simulink model "Trapezoidal_Commutation_BLDC_Motor_2024b"  (R2024b)
settings: Solver=VariableStepAuto  StartTime=0.0  StopTime=2  RelTol=1e-3
libraries: nesl_utility x11, ee_lib x10, fl_lib x6
settings Model: LastModifiedBy=Ashwin VJ
settings ConfigComp: CovBoundaryAbsTol=1.0e-5

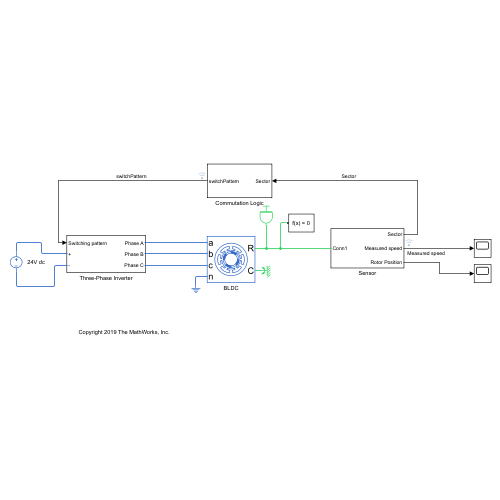
[thumbnail: Simulink's stored preview of the top-level diagram]
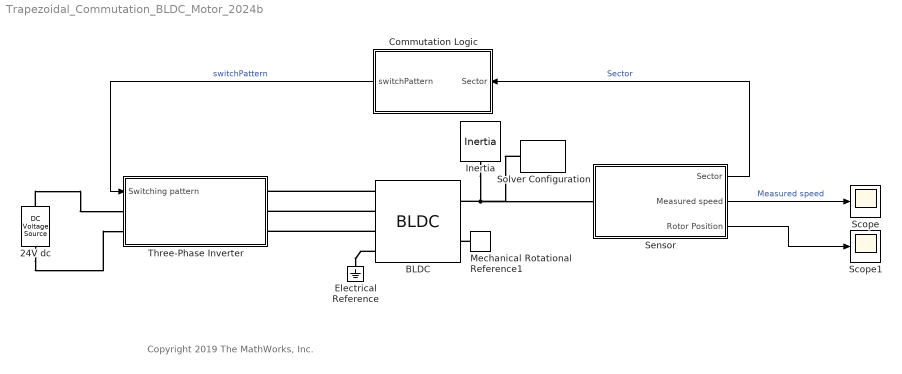
== system Trapezoidal_Commutation_BLDC_Motor_2024b ==
  note: Copyright 2019 The MathWorks, Inc.
  24V dc : ee_lib/Additional Components/SPICE Sources/DC Voltage Source  DC=24 V
  BLDC : ee_lib/Electromechanical/Permanent Magnet/BLDC  port_option=ee.enum.threePhasePort.expanded  rotor_param=1  pm_flux_linkage=0.55 Wb  theta_constant=120/1 deg  emf_max=9.6 V  w_meas=600 rpm  DphiDtheta_tab=[0, -.1528, -.1528, .1528, .1528, 0] Wb/rad  back_emf_tab=[0, -9.6, -9.6, 9.6, 9.6, 0] V  rotor_angle_tab=[0, 7.5, 22.5, 37.5, 52.5, 60] deg  nPolePairs=1  axes_param=1  winding_type=ee.enum.statorconnection.wye  stator_param=ee.enum.statorparam.LdLqL0  machine_param=ee.enum.dqparameterization.constant  Ld=0.00022 H  Lq=0.00022 H  idVec=[-200, 0, 200] A  iqVec=[-200, 0, 200] A  LdMatrix=0.00022 * ones(3, 3) H  LqMatrix=0.00022 * ones(3, 3) H  L0=0.00022 H  Ls=0.0002 H  Lm=0 H  Ms=0.00002 H  Rs=0.13 Ohm  zero_sequence=ee.enum.park.zerosequence.include  loss_param=ee.enum.ironloss.none  losses_oc=[0, 0, 0] W  losses_sc=[0, 0, 0] W  f_losses=60 Hz  Isc_losses=95 A  J=0.0001 kg*m^2  lam=0.2 N*m/(rad/s)  i_d_specify=off  i_d_priority=None  i_d=0 A  i_d_nominal_specify=off  i_d_nominal_value=1  i_d_nominal_unit=A  i_q_specify=off  i_q_priority=None  i_q=0 A  i_q_nominal_specify=off  i_q_nominal_value=1  i_q_nominal_unit=A  torque_specify=off  torque_priority=None  torque=0 N*m  torque_nominal_specify=off  torque_nominal_value=1  torque_nominal_unit=N*m  angular_velocity_specify=off  angular_velocity_priority=High  angular_velocity=0 rpm  angular_velocity_nominal_specify=off  angular_velocity_nominal_value=1  angular_velocity_nominal_unit=rpm  angular_position_specify=off  angular_position_priority=High  angular_position=0 deg  angular_position_nominal_specify=off  angular_position_nominal_value=1  angular_position_nominal_unit=deg  alpha=3.93e-3 1/K  alpha_flux=-0.001 1/K  Tmeas=298.15 K  stator_thermal_mass=100 J/K  rotor_thermal_mass=200 J/K  Rm_percent_rotor=90  Rd_percent_rotor=30  temperatureA_specify=off  temperatureA_priority=High  temperatureA=25 degC  temperatureA_nominal_specify=off  temperatureA_nominal_value=1  temperatureA_nominal_unit=degC  temperatureB_specify=off  temperatureB_priority=High  temperatureB=25 degC  temperatureB_nominal_specify=off  temperatureB_nominal_value=1  temperatureB_nominal_unit=degC  temperatureC_specify=off  temperatureC_priority=High  temperatureC=25 degC  temperatureC_nominal_specify=off  temperatureC_nominal_value=1  temperatureC_nominal_unit=degC  temperatureR_specify=off  temperatureR_priority=High  temperatureR=25 degC  temperatureR_nominal_specify=off  temperatureR_nominal_value=1  temperatureR_nominal_unit=degC
      settings: InternalSimscapePortConfiguration="{\"Bottom\":[],\"Left\":[{\"id\":\"a\",\"label\":\"a\",\"type\":\"foundation.electrical.electrical\"},{\"id\":\"b\",\"label\":\"b\",\"type\":\"foundation.electrical.electrical\"},{\"id\":\"c\",\"label\":\"c\",\"type\":\"foundation.electrical.electrical\"},{\"id\":\"n\",\"label\":\"n\",\"type\":\"foundation.electrical.electrical\"}],\"Right\":[{\"id\":\"R\",\"label\":\"R\",\"type\":\"foundation.mechanical.rotational.rotational\"},{\"id\":\"C\",\"label\":\"C\",\"type\":\"foundation.mechanical.rotational.rotational\"}],\"Top\":[]}"
  Commutation Logic : Subsystem
  Electrical Reference : fl_lib/Electrical/Electrical Elements/Electrical Reference
  Inertia : fl_lib/Mechanical/Rotational Elements/Inertia  inertia=0.2 kg*m^2  num_ports=foundation.enum.numPorts2.one  w_specify=off  w_priority=High  w=0 rad/s  w_nominal_specify=off  w_nominal_value=1  w_nominal_unit=rad/s  t_specify=off  t_priority=None  t=0 N*m  t_nominal_specify=off  t_nominal_value=1  t_nominal_unit=N*m
  Mechanical Rotational Reference1 : fl_lib/Mechanical/Rotational Elements/Mechanical Rotational Reference
  Scope : Scope
  Scope1 : Scope
  Sensor : Subsystem
  Solver Configuration : nesl_utility/Solver Configuration  PhysicalDomain=network_engine_domain  SubClassName=solver  LeftPortType=input  RightPortType=generic  Tones=[]  Harmonics=[]  SimulateNoise=off  Profile=off  UseLocalSampling=off  EnableSwitchedLinearOptims=on  FrequencyDomain=off  UseCCode=off  RelTol=0.001  AbsTol=1e-06  MinStep=1e-09  ToWorkspace=off  RevertToSquareIcSolve=off  NumHomotopyIterations=100  PhasorMode=off  PhasorModeNumHarmonics=1  ConsistencySolver=NEWTON_FTOL  IndexReductionMethod=DerivativeReplacement  DoDC=off  ResidualTolerance=1e-09  ConsistencyTolSource=GLOBAL  ConsistencyAbsTol=0.001  ConsistencyRelTol=0.001  ConsistencyTolFactor=0.001  UseLocalSolver=on  LocalSolverChoice=NE_BACKWARD_EULER_ADVANCER  ResolveIndetEquations=on  FunctionEvalNumThread=1  LocalSolverSampleTime=2e-5  DoFixedCost=on  MaxNonlinIter=4  MaxModeIter=2  ComputeImpulses=off  ImpulseIterations=2  LinearAlgebra=auto  LinearAlgebraNumThread=0  EquationFormulation=NE_TIME_EF  DelaysMemoryBudget=1024  AutomaticFiltering=off  FilteringTimeConstant=0.001  PartitionStorageMethod=AS_NEEDED  PartitionMemoryBudget=1024  PartitionMethod=ROBUST  MultibodyUseLocalSolver=off  MultibodyLocalSolverChoice=ODE1  MultibodyLocalSolverSampleTime=0.001
  Three-Phase Inverter : Subsystem
  wires:
  Sensor/1(Sector) -> Commutation Logic/1(Sector)  "Sector"
  Commutation Logic/1(switchPattern) -> Three-Phase Inverter/1(Switching pattern)  "switchPattern"
  Sensor/2(Measured speed) -> Scope/1  "Measured speed"
  Sensor/3(Rotor Position) -> Scope1/1
  connections:
  Inertia/LConn1 -- Solver Configuration/RConn1 -- Sensor/LConn1 -- BLDC/RConn1
  Mechanical Rotational Reference1/LConn1 -- BLDC/RConn2
  BLDC/LConn2 -- Three-Phase Inverter/RConn2
  BLDC/LConn4 -- Electrical Reference/LConn1
  BLDC/LConn1 -- Three-Phase Inverter/RConn1
  BLDC/LConn3 -- Three-Phase Inverter/RConn3
  24V dc/LConn1 -- Three-Phase Inverter/LConn1
  24V dc/RConn1 -- Three-Phase Inverter/LConn2

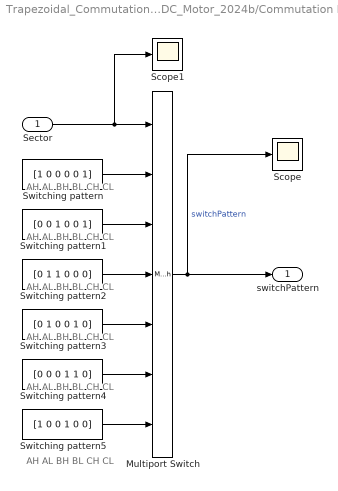
== system Trapezoidal_Commutation_BLDC_Motor_2024b/Commutation Logic ==
  note: AH AL BH BL CH CL
  note: AH AL BH BL CH CL
  note: AH AL BH BL CH CL
  note: AH AL BH BL CH CL
  note: AH AL BH BL CH CL
  note: AH AL BH BL CH CL
  Sector : Inport
  Multiport Switch : MultiPortSwitch  Inputs=6  SaturateOnIntegerOverflow=off  InputSameDT=off
  Scope : Scope
  Scope1 : Scope
  Switching pattern : Constant  Value=[1 0 0 0 0 1]
  Switching pattern1 : Constant  Value=[0 0 1 0 0 1]
  Switching pattern2 : Constant  Value=[0 1 1 0 0 0]
  Switching pattern3 : Constant  Value=[0 1 0 0 1 0]
  Switching pattern4 : Constant  Value=[0 0 0 1 1 0]
  Switching pattern5 : Constant  Value=[1 0 0 1 0 0]
  switchPattern : Outport
  wires:
  Switching pattern3/1 -> Multiport Switch/5
  Switching pattern2/1 -> Multiport Switch/4
  Multiport Switch/1 -> Scope/1, switchPattern/1  "switchPattern"
  Switching pattern1/1 -> Multiport Switch/3
  Switching pattern5/1 -> Multiport Switch/7
  Sector/1 -> Scope1/1, Multiport Switch/1
  Switching pattern4/1 -> Multiport Switch/6
  Switching pattern/1 -> Multiport Switch/2

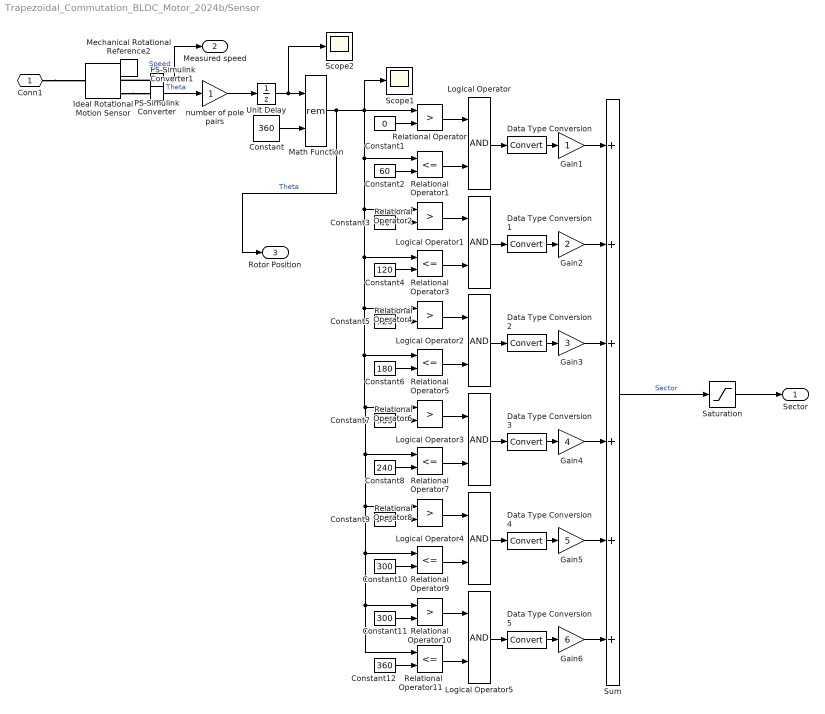
== system Trapezoidal_Commutation_BLDC_Motor_2024b/Sensor ==
  Constant : Constant  Value=360
  Constant1 : Constant  Value=0
  Constant10 : Constant  Value=300
  Constant11 : Constant  Value=300
  Constant12 : Constant  Value=360
  Constant2 : Constant  Value=60
  Constant3 : Constant  Value=60
  Constant4 : Constant  Value=120
  Constant5 : Constant  Value=120
  Constant6 : Constant  Value=180
  Constant7 : Constant  Value=180
  Constant8 : Constant  Value=240
  Constant9 : Constant  Value=240
  Data Type Conversion{,1..5} (6 alike) : DataTypeConversion  SaturateOnIntegerOverflow=off  RndMeth=Floor
  Gain1 : Gain
  Gain2 : Gain  Gain=2
  Gain3 : Gain  Gain=3
  Gain4 : Gain  Gain=4
  Gain5 : Gain  Gain=5
  Gain6 : Gain  Gain=6
  Ideal Rotational Motion Sensor : fl_lib/Mechanical/Mechanical Sensors/Ideal Rotational Motion Sensor  reference=foundation.enum.MeasurementReference.difference  acceleration_port=false  velocity_port=true  position_port=true  wrap_angle=false  offset=0 deg
  Logical Operator{,1..5} (6 alike) : Logic  AllPortsSameDT=off  OutDataTypeStr=boolean
  Math Function : Math  Operator=rem
  Mechanical Rotational Reference2 : fl_lib/Mechanical/Rotational Elements/Mechanical Rotational Reference
  PS-Simulink Converter : nesl_utility/PS-Simulink Converter  PhysicalDomain=network_engine_domain  SubClassName=ps_output  LeftPortType=input  RightPortType=output  PseudoPeriodic=off  Frequencies=[]  VectorFormat=1-D array  Unit=rpm  AffineConversion=off
  PS-Simulink Converter1 : nesl_utility/PS-Simulink Converter  PhysicalDomain=network_engine_domain  SubClassName=ps_output  LeftPortType=input  RightPortType=output  PseudoPeriodic=off  Frequencies=[]  VectorFormat=1-D array  Unit=deg  AffineConversion=off
  Relational Operator{,2,4,6,8,10} (6 alike) : RelationalOperator  Operator=>  OutDataTypeStr=boolean  RndMeth=Simplest  InputSameDT=off
  Relational Operator{1,3,5,7,9,11} (6 alike) : RelationalOperator  Operator=<=  OutDataTypeStr=boolean  RndMeth=Simplest  InputSameDT=off
  Saturation : Saturate  UpperLimit=6  LowerLimit=1
  Scope1 : Scope
  Scope2 : Scope
  Sum : Sum  Inputs=++++++
  Unit Delay : UnitDelay  SampleTime=2e-5  HasFrameUpgradeWarning=on
  number of pole pairs : Gain
  Conn1 : PMIOPort  Side=Left
  Sector : Outport
  Measured speed : Outport  Port=2
  Rotor Position : Outport  Port=3
  wires:
  Math Function/1 -> Scope1/1, Relational Operator11/1, Relational Operator10/1, Relational Operator9/1, Relational Operator8/1, Relational Operator7/1, Relational Operator6/1, Relational Operator5/1, Relational Operator4/1, Relational Operator3/1, Relational Operator2/1, Relational Operator1/1, Relational Operator/1, Rotor Position/1  "Theta"
  Relational Operator9/1 -> Logical Operator4/2
  Relational Operator/1 -> Logical Operator/1
  Constant9/1 -> Relational Operator8/2
  Relational Operator2/1 -> Logical Operator1/1
  Constant7/1 -> Relational Operator6/2
  Relational Operator10/1 -> Logical Operator5/1
  Constant/1 -> Math Function/2
  Logical Operator5/1 -> Data Type Conversion5/1
  Relational Operator6/1 -> Logical Operator3/1
  Logical Operator/1 -> Data Type Conversion/1
  Constant11/1 -> Relational Operator10/2
  Data Type Conversion4/1 -> Gain5/1
  Constant10/1 -> Relational Operator9/2
  Constant12/1 -> Relational Operator11/2
  Relational Operator3/1 -> Logical Operator1/2
  PS-Simulink Converter1/1 -> number of pole pairs/1  "Theta"
  Logical Operator4/1 -> Data Type Conversion4/1
  Relational Operator5/1 -> Logical Operator2/2
  PS-Simulink Converter/1 -> Measured speed/1  "Speed"
  Data Type Conversion3/1 -> Gain4/1
  Gain2/1 -> Sum/2
  Gain6/1 -> Sum/6
  Relational Operator1/1 -> Logical Operator/2
  Data Type Conversion5/1 -> Gain6/1
  Data Type Conversion/1 -> Gain1/1
  Unit Delay/1 -> Scope2/1, Math Function/1
  Gain4/1 -> Sum/4
  Constant1/1 -> Relational Operator/2
  Gain3/1 -> Sum/3
  Relational Operator11/1 -> Logical Operator5/2
  Constant2/1 -> Relational Operator1/2
  Constant6/1 -> Relational Operator5/2
  Constant8/1 -> Relational Operator7/2
  Relational Operator4/1 -> Logical Operator2/1
  Relational Operator8/1 -> Logical Operator4/1
  Constant3/1 -> Relational Operator2/2
  Relational Operator7/1 -> Logical Operator3/2
  Data Type Conversion2/1 -> Gain3/1
  number of pole pairs/1 -> Unit Delay/1
  Data Type Conversion1/1 -> Gain2/1
  Logical Operator2/1 -> Data Type Conversion2/1
  Logical Operator1/1 -> Data Type Conversion1/1
  Logical Operator3/1 -> Data Type Conversion3/1
  Gain5/1 -> Sum/5
  Constant4/1 -> Relational Operator3/2
  Constant5/1 -> Relational Operator4/2
  Gain1/1 -> Sum/1
  Sum/1 -> Saturation/1  "Sector"
  Saturation/1 -> Sector/1
  connections:
  Ideal Rotational Motion Sensor/RConn3 -- PS-Simulink Converter1/LConn1
  PS-Simulink Converter/LConn1 -- Ideal Rotational Motion Sensor/RConn2
  Mechanical Rotational Reference2/LConn1 -- Ideal Rotational Motion Sensor/RConn1
  Conn1/RConn1 -- Ideal Rotational Motion Sensor/LConn1

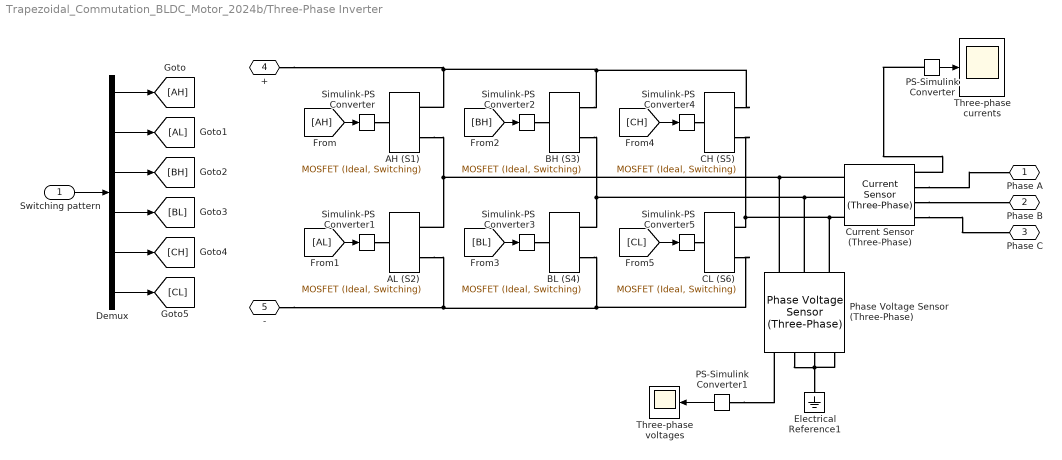
== system Trapezoidal_Commutation_BLDC_Motor_2024b/Three-Phase Inverter ==
  Switching pattern : Inport
  AH (S1) : ee_lib/Semiconductors & Converters/MOSFET (Ideal, Switching)  port_option=ee.enum.controlport.ps  Rds=0.01 Ohm  Goff=1e-6 1/Ohm  Vth=0.5 V  diode_param=2  diode_Vf=0.1 V  diode_Ron=0.001 Ohm  diode_Goff=1e-5 1/Ohm  diode_C=50e-9 F  diode_iRM=-235 A  diode_iF=300 A  diode_idot=-50 A/us  diode_trr_param=1  diode_trr_factor=3  diode_trr=15 us  diode_Qrr=1500 s*uA  ids_specify=off  ids_priority=None  ids=0 A  ids_nominal_specify=off  ids_nominal_value=1  ids_nominal_unit=A  vds_specify=off  vds_priority=None  vds=0 V  vds_nominal_specify=off  vds_nominal_value=1  vds_nominal_unit=V  vgs_specify=off  vgs_priority=None  vgs=0 V  vgs_nominal_specify=off  vgs_nominal_value=1  vgs_nominal_unit=V  thermal_loss_option=2  Von_data=[0, 1.1, 1.3, 1.45, 1.75, 2.25, 2.7; 0, 1, 1.15, 1.35, 1.7, 2.35, 3] V  Tj=[298.15, 398.15] K  Iout_data=[0, 10, 50, 100, 200, 400, 600] A  Eon_data=[0, .29, 1.43, 2.86, 5.71, 13.14, 22.86; 0, .57, 2.63, 5.14, 10.29, 20.57, 30.29] * 1e-3 J  Eoff_data=[0, .21, 1.07, 2.14, 4.29, 9.86, 17.14; 0, .43, 1.97, 3.86, 7.71, 15.43, 22.71] * 1e-3 J  Eon_data_3D=[zeros(2, 5, 3)] J  Eoff_data_3D=[zeros(2, 5, 3)] J  Tj_loss=[298.15, 448.15] K  Iout_data_loss=[0, 10, 20, 30, 40] A  tabulateWithVds=false  Vds_loss=[0, 150, 300] V  Eon_scalar=22.86e-3 J  Eoff_scalar=17.14e-3 J  Voff=300 V  Iout_scalar=600 A  useCurrentFromPreviousCycle=false  useVoltageFromPreviousCycle=false  diodeModelType=ee.enum.converters.diodeModelType.pwl  diodeTableType=ee.enum.diode.tableType.IfMat  diode_ReverseIVType=ee.enum.diode.diodeReverseIV.constant  diode_IfMat=[.07, .12, .19, 1.75, 4.24, 7.32, 11.2; .16, .3, .72, 2.14, 4.02, 6.35, 9.12] A  diode_VfMat=[.9, 1.15, 1.25, 1.5, 1.75, 2.17, 2.6, 2.85; .58, .68, .75, 1.1, 1.38, 1.77, 2.27, 2.7] V  diode_TjVec=[25, 125] degC  diode_VfVec=[.5, .7, .9, 1.3, 1.7, 2.1, 2.5] V  diode_IfVec=[.1, .2, .5, 1, 2, 4, 7, 10] A  diode_IrMat=[1e-06, 2e-06, 5e-06, 1e-05, 2.5e-05, 5e-05, .0001; 2e-06, 5e-06, 1e-05, 4e-05, 8e-05, .0002, .0005] A  diode_VrMat=[10, 100, 200, 250, 300, 325, 350; 10, 70, 160, 220, 270, 300, 320] V  diode_VrVec=[10, 20, 40, 50, 70, 80, 100] V  diode_IrVec=[1e-06, 2e-06, 5e-06, 1e-05, 2e-05, 5e-05, .0001] A  diode_Vr=-600 V  diode_Ls=150 nH  diode_Erec=0.03 J  diode_rec_loss_model=ee.enum.diode.reverseRecoveryModel.fixed  diode_ErecVal=0 J  diode_scaleWithIandV=true  diode_ErecMat=zeros(2, 3) J  diode_TjrecVec=[298.15, 398.15] K  diode_IfrecVec=[.1, 1, 10] A  diode_IrecVal=10 A  diode_VrecVal=10 V  diode_tFilter=1 / 1000 / 100 s  separateThermalPortForDiode=false  thermal_network_parameterization=ee.enum.thermalNetworkTopology.external  Rth=[.03, .2] K/W  Rth_Cauer=[.03, .1, .2] K/W  Rth_Foster=[.03, .2] K/W  thermal_mass_parameterization=ee.enum.thermalNetwork.timeconstant  thermal_mass=[3, 25] J/K  thermal_mass_Cauer=[3, 10, 25] J/K  thermal_mass_Foster=[33, 50] J/K  thermal_time_constant=[.1, 5] s  thermal_time_constant_Cauer=[.1, 1, 5] s  thermal_time_constant_Foster=[1, 10] s  thermal_mass_initial_temperatures=[25, 25] degC  thermal_mass_initial_temperatures_Cauer=[25, 25, 25] degC  junction_thermal_mass=0.1 J/K  Tvec_initial_Foster=[25, 25, 25, 25] degC  RthDiode=[.03, .2] K/W  RthCauerDiode=[.03, .1, .2] K/W  RthFosterDiode=[.03, .2] K/W  thermalMassDiode=[3, 25] J/K  thermalMassCauerDiode=[3, 10, 25] J/K  thermalMassFosterDiode=[33, 50] J/K  thermalTauDiode=[.1, 5] s  thermalTauCauerDiode=[.1, 1, 5] s  thermalTauFosterDiode=[1, 10] s  thermalMassInitTempDiode=[25, 25] degC  thermalMassInitTempCauerDiode=[25, 25, 25] degC  junctionthermalMassDiode=0.1 J/K  TVecInitialFosterDiode=[25, 25, 25, 25] degC  no_thermal_network=0  mosfet_junction_temperature_specify=off  mosfet_junction_temperature_priority=None  mosfet_junction_temperature=25 degC  mosfet_junction_temperature_nominal_specify=off  mosfet_junction_temperature_nominal_value=1  mosfet_junction_temperature_nominal_unit=degC  diode_junction_temperature_specify=off  diode_junction_temperature_priority=None  diode_junction_temperature=25 degC  diode_junction_temperature_nominal_specify=off  diode_junction_temperature_nominal_value=1  diode_junction_temperature_nominal_unit=degC  Qj_specify=off  Qj_priority=None  Qj=0 W  Qj_nominal_specify=off  Qj_nominal_value=1  Qj_nominal_unit=W  accumulatedSwitchingLosses_specify=off  accumulatedSwitchingLosses_priority=None  accumulatedSwitchingLosses=0 J
  AL (S2) : ee_lib/Semiconductors & Converters/MOSFET (Ideal, Switching)  port_option=ee.enum.controlport.ps  Rds=0.01 Ohm  Goff=1e-6 1/Ohm  Vth=0.5 V  diode_param=2  diode_Vf=0.1 V  diode_Ron=0.001 Ohm  diode_Goff=1e-5 1/Ohm  diode_C=50e-9 F  diode_iRM=-235 A  diode_iF=300 A  diode_idot=-50 A/us  diode_trr_param=1  diode_trr_factor=3  diode_trr=15 us  diode_Qrr=1500 s*uA  ids_specify=off  ids_priority=None  ids=0 A  ids_nominal_specify=off  ids_nominal_value=1  ids_nominal_unit=A  vds_specify=off  vds_priority=None  vds=0 V  vds_nominal_specify=off  vds_nominal_value=1  vds_nominal_unit=V  vgs_specify=off  vgs_priority=None  vgs=0 V  vgs_nominal_specify=off  vgs_nominal_value=1  vgs_nominal_unit=V  thermal_loss_option=2  Von_data=[0, 1.1, 1.3, 1.45, 1.75, 2.25, 2.7; 0, 1, 1.15, 1.35, 1.7, 2.35, 3] V  Tj=[298.15, 398.15] K  Iout_data=[0, 10, 50, 100, 200, 400, 600] A  Eon_data=[0, .29, 1.43, 2.86, 5.71, 13.14, 22.86; 0, .57, 2.63, 5.14, 10.29, 20.57, 30.29] * 1e-3 J  Eoff_data=[0, .21, 1.07, 2.14, 4.29, 9.86, 17.14; 0, .43, 1.97, 3.86, 7.71, 15.43, 22.71] * 1e-3 J  Eon_data_3D=[zeros(2, 5, 3)] J  Eoff_data_3D=[zeros(2, 5, 3)] J  Tj_loss=[298.15, 448.15] K  Iout_data_loss=[0, 10, 20, 30, 40] A  tabulateWithVds=false  Vds_loss=[0, 150, 300] V  Eon_scalar=22.86e-3 J  Eoff_scalar=17.14e-3 J  Voff=300 V  Iout_scalar=600 A  useCurrentFromPreviousCycle=false  useVoltageFromPreviousCycle=false  diodeModelType=ee.enum.converters.diodeModelType.pwl  diodeTableType=ee.enum.diode.tableType.IfMat  diode_ReverseIVType=ee.enum.diode.diodeReverseIV.constant  diode_IfMat=[.07, .12, .19, 1.75, 4.24, 7.32, 11.2; .16, .3, .72, 2.14, 4.02, 6.35, 9.12] A  diode_VfMat=[.9, 1.15, 1.25, 1.5, 1.75, 2.17, 2.6, 2.85; .58, .68, .75, 1.1, 1.38, 1.77, 2.27, 2.7] V  diode_TjVec=[25, 125] degC  diode_VfVec=[.5, .7, .9, 1.3, 1.7, 2.1, 2.5] V  diode_IfVec=[.1, .2, .5, 1, 2, 4, 7, 10] A  diode_IrMat=[1e-06, 2e-06, 5e-06, 1e-05, 2.5e-05, 5e-05, .0001; 2e-06, 5e-06, 1e-05, 4e-05, 8e-05, .0002, .0005] A  diode_VrMat=[10, 100, 200, 250, 300, 325, 350; 10, 70, 160, 220, 270, 300, 320] V  diode_VrVec=[10, 20, 40, 50, 70, 80, 100] V  diode_IrVec=[1e-06, 2e-06, 5e-06, 1e-05, 2e-05, 5e-05, .0001] A  diode_Vr=-600 V  diode_Ls=150 nH  diode_Erec=0.03 J  diode_rec_loss_model=ee.enum.diode.reverseRecoveryModel.fixed  diode_ErecVal=0 J  diode_scaleWithIandV=true  diode_ErecMat=zeros(2, 3) J  diode_TjrecVec=[298.15, 398.15] K  diode_IfrecVec=[.1, 1, 10] A  diode_IrecVal=10 A  diode_VrecVal=10 V  diode_tFilter=1 / 1000 / 100 s  separateThermalPortForDiode=false  thermal_network_parameterization=ee.enum.thermalNetworkTopology.external  Rth=[.03, .2] K/W  Rth_Cauer=[.03, .1, .2] K/W  Rth_Foster=[.03, .2] K/W  thermal_mass_parameterization=ee.enum.thermalNetwork.timeconstant  thermal_mass=[3, 25] J/K  thermal_mass_Cauer=[3, 10, 25] J/K  thermal_mass_Foster=[33, 50] J/K  thermal_time_constant=[.1, 5] s  thermal_time_constant_Cauer=[.1, 1, 5] s  thermal_time_constant_Foster=[1, 10] s  thermal_mass_initial_temperatures=[25, 25] degC  thermal_mass_initial_temperatures_Cauer=[25, 25, 25] degC  junction_thermal_mass=0.1 J/K  Tvec_initial_Foster=[25, 25, 25, 25] degC  RthDiode=[.03, .2] K/W  RthCauerDiode=[.03, .1, .2] K/W  RthFosterDiode=[.03, .2] K/W  thermalMassDiode=[3, 25] J/K  thermalMassCauerDiode=[3, 10, 25] J/K  thermalMassFosterDiode=[33, 50] J/K  thermalTauDiode=[.1, 5] s  thermalTauCauerDiode=[.1, 1, 5] s  thermalTauFosterDiode=[1, 10] s  thermalMassInitTempDiode=[25, 25] degC  thermalMassInitTempCauerDiode=[25, 25, 25] degC  junctionthermalMassDiode=0.1 J/K  TVecInitialFosterDiode=[25, 25, 25, 25] degC  no_thermal_network=0  mosfet_junction_temperature_specify=off  mosfet_junction_temperature_priority=None  mosfet_junction_temperature=25 degC  mosfet_junction_temperature_nominal_specify=off  mosfet_junction_temperature_nominal_value=1  mosfet_junction_temperature_nominal_unit=degC  diode_junction_temperature_specify=off  diode_junction_temperature_priority=None  diode_junction_temperature=25 degC  diode_junction_temperature_nominal_specify=off  diode_junction_temperature_nominal_value=1  diode_junction_temperature_nominal_unit=degC  Qj_specify=off  Qj_priority=None  Qj=0 W  Qj_nominal_specify=off  Qj_nominal_value=1  Qj_nominal_unit=W  accumulatedSwitchingLosses_specify=off  accumulatedSwitchingLosses_priority=None  accumulatedSwitchingLosses=0 J
  BH (S3) : ee_lib/Semiconductors & Converters/MOSFET (Ideal, Switching)  port_option=ee.enum.controlport.ps  Rds=0.01 Ohm  Goff=1e-6 1/Ohm  Vth=0.5 V  diode_param=2  diode_Vf=0.1 V  diode_Ron=0.001 Ohm  diode_Goff=1e-5 1/Ohm  diode_C=50e-9 F  diode_iRM=-235 A  diode_iF=300 A  diode_idot=-50 A/us  diode_trr_param=1  diode_trr_factor=3  diode_trr=15 us  diode_Qrr=1500 s*uA  ids_specify=off  ids_priority=None  ids=0 A  ids_nominal_specify=off  ids_nominal_value=1  ids_nominal_unit=A  vds_specify=off  vds_priority=None  vds=0 V  vds_nominal_specify=off  vds_nominal_value=1  vds_nominal_unit=V  vgs_specify=off  vgs_priority=None  vgs=0 V  vgs_nominal_specify=off  vgs_nominal_value=1  vgs_nominal_unit=V  thermal_loss_option=2  Von_data=[0, 1.1, 1.3, 1.45, 1.75, 2.25, 2.7; 0, 1, 1.15, 1.35, 1.7, 2.35, 3] V  Tj=[298.15, 398.15] K  Iout_data=[0, 10, 50, 100, 200, 400, 600] A  Eon_data=[0, .29, 1.43, 2.86, 5.71, 13.14, 22.86; 0, .57, 2.63, 5.14, 10.29, 20.57, 30.29] * 1e-3 J  Eoff_data=[0, .21, 1.07, 2.14, 4.29, 9.86, 17.14; 0, .43, 1.97, 3.86, 7.71, 15.43, 22.71] * 1e-3 J  Eon_data_3D=[zeros(2, 5, 3)] J  Eoff_data_3D=[zeros(2, 5, 3)] J  Tj_loss=[298.15, 448.15] K  Iout_data_loss=[0, 10, 20, 30, 40] A  tabulateWithVds=false  Vds_loss=[0, 150, 300] V  Eon_scalar=22.86e-3 J  Eoff_scalar=17.14e-3 J  Voff=300 V  Iout_scalar=600 A  useCurrentFromPreviousCycle=false  useVoltageFromPreviousCycle=false  diodeModelType=ee.enum.converters.diodeModelType.pwl  diodeTableType=ee.enum.diode.tableType.IfMat  diode_ReverseIVType=ee.enum.diode.diodeReverseIV.constant  diode_IfMat=[.07, .12, .19, 1.75, 4.24, 7.32, 11.2; .16, .3, .72, 2.14, 4.02, 6.35, 9.12] A  diode_VfMat=[.9, 1.15, 1.25, 1.5, 1.75, 2.17, 2.6, 2.85; .58, .68, .75, 1.1, 1.38, 1.77, 2.27, 2.7] V  diode_TjVec=[25, 125] degC  diode_VfVec=[.5, .7, .9, 1.3, 1.7, 2.1, 2.5] V  diode_IfVec=[.1, .2, .5, 1, 2, 4, 7, 10] A  diode_IrMat=[1e-06, 2e-06, 5e-06, 1e-05, 2.5e-05, 5e-05, .0001; 2e-06, 5e-06, 1e-05, 4e-05, 8e-05, .0002, .0005] A  diode_VrMat=[10, 100, 200, 250, 300, 325, 350; 10, 70, 160, 220, 270, 300, 320] V  diode_VrVec=[10, 20, 40, 50, 70, 80, 100] V  diode_IrVec=[1e-06, 2e-06, 5e-06, 1e-05, 2e-05, 5e-05, .0001] A  diode_Vr=-600 V  diode_Ls=150 nH  diode_Erec=0.03 J  diode_rec_loss_model=ee.enum.diode.reverseRecoveryModel.fixed  diode_ErecVal=0 J  diode_scaleWithIandV=true  diode_ErecMat=zeros(2, 3) J  diode_TjrecVec=[298.15, 398.15] K  diode_IfrecVec=[.1, 1, 10] A  diode_IrecVal=10 A  diode_VrecVal=10 V  diode_tFilter=1 / 1000 / 100 s  separateThermalPortForDiode=false  thermal_network_parameterization=ee.enum.thermalNetworkTopology.external  Rth=[.03, .2] K/W  Rth_Cauer=[.03, .1, .2] K/W  Rth_Foster=[.03, .2] K/W  thermal_mass_parameterization=ee.enum.thermalNetwork.timeconstant  thermal_mass=[3, 25] J/K  thermal_mass_Cauer=[3, 10, 25] J/K  thermal_mass_Foster=[33, 50] J/K  thermal_time_constant=[.1, 5] s  thermal_time_constant_Cauer=[.1, 1, 5] s  thermal_time_constant_Foster=[1, 10] s  thermal_mass_initial_temperatures=[25, 25] degC  thermal_mass_initial_temperatures_Cauer=[25, 25, 25] degC  junction_thermal_mass=0.1 J/K  Tvec_initial_Foster=[25, 25, 25, 25] degC  RthDiode=[.03, .2] K/W  RthCauerDiode=[.03, .1, .2] K/W  RthFosterDiode=[.03, .2] K/W  thermalMassDiode=[3, 25] J/K  thermalMassCauerDiode=[3, 10, 25] J/K  thermalMassFosterDiode=[33, 50] J/K  thermalTauDiode=[.1, 5] s  thermalTauCauerDiode=[.1, 1, 5] s  thermalTauFosterDiode=[1, 10] s  thermalMassInitTempDiode=[25, 25] degC  thermalMassInitTempCauerDiode=[25, 25, 25] degC  junctionthermalMassDiode=0.1 J/K  TVecInitialFosterDiode=[25, 25, 25, 25] degC  no_thermal_network=0  mosfet_junction_temperature_specify=off  mosfet_junction_temperature_priority=None  mosfet_junction_temperature=25 degC  mosfet_junction_temperature_nominal_specify=off  mosfet_junction_temperature_nominal_value=1  mosfet_junction_temperature_nominal_unit=degC  diode_junction_temperature_specify=off  diode_junction_temperature_priority=None  diode_junction_temperature=25 degC  diode_junction_temperature_nominal_specify=off  diode_junction_temperature_nominal_value=1  diode_junction_temperature_nominal_unit=degC  Qj_specify=off  Qj_priority=None  Qj=0 W  Qj_nominal_specify=off  Qj_nominal_value=1  Qj_nominal_unit=W  accumulatedSwitchingLosses_specify=off  accumulatedSwitchingLosses_priority=None  accumulatedSwitchingLosses=0 J
  BL (S4) : ee_lib/Semiconductors & Converters/MOSFET (Ideal, Switching)  port_option=ee.enum.controlport.ps  Rds=0.01 Ohm  Goff=1e-6 1/Ohm  Vth=0.5 V  diode_param=2  diode_Vf=0.1 V  diode_Ron=0.001 Ohm  diode_Goff=1e-5 1/Ohm  diode_C=50e-9 F  diode_iRM=-235 A  diode_iF=300 A  diode_idot=-50 A/us  diode_trr_param=1  diode_trr_factor=3  diode_trr=15 us  diode_Qrr=1500 s*uA  ids_specify=off  ids_priority=None  ids=0 A  ids_nominal_specify=off  ids_nominal_value=1  ids_nominal_unit=A  vds_specify=off  vds_priority=None  vds=0 V  vds_nominal_specify=off  vds_nominal_value=1  vds_nominal_unit=V  vgs_specify=off  vgs_priority=None  vgs=0 V  vgs_nominal_specify=off  vgs_nominal_value=1  vgs_nominal_unit=V  thermal_loss_option=2  Von_data=[0, 1.1, 1.3, 1.45, 1.75, 2.25, 2.7; 0, 1, 1.15, 1.35, 1.7, 2.35, 3] V  Tj=[298.15, 398.15] K  Iout_data=[0, 10, 50, 100, 200, 400, 600] A  Eon_data=[0, .29, 1.43, 2.86, 5.71, 13.14, 22.86; 0, .57, 2.63, 5.14, 10.29, 20.57, 30.29] * 1e-3 J  Eoff_data=[0, .21, 1.07, 2.14, 4.29, 9.86, 17.14; 0, .43, 1.97, 3.86, 7.71, 15.43, 22.71] * 1e-3 J  Eon_data_3D=[zeros(2, 5, 3)] J  Eoff_data_3D=[zeros(2, 5, 3)] J  Tj_loss=[298.15, 448.15] K  Iout_data_loss=[0, 10, 20, 30, 40] A  tabulateWithVds=false  Vds_loss=[0, 150, 300] V  Eon_scalar=22.86e-3 J  Eoff_scalar=17.14e-3 J  Voff=300 V  Iout_scalar=600 A  useCurrentFromPreviousCycle=false  useVoltageFromPreviousCycle=false  diodeModelType=ee.enum.converters.diodeModelType.pwl  diodeTableType=ee.enum.diode.tableType.IfMat  diode_ReverseIVType=ee.enum.diode.diodeReverseIV.constant  diode_IfMat=[.07, .12, .19, 1.75, 4.24, 7.32, 11.2; .16, .3, .72, 2.14, 4.02, 6.35, 9.12] A  diode_VfMat=[.9, 1.15, 1.25, 1.5, 1.75, 2.17, 2.6, 2.85; .58, .68, .75, 1.1, 1.38, 1.77, 2.27, 2.7] V  diode_TjVec=[25, 125] degC  diode_VfVec=[.5, .7, .9, 1.3, 1.7, 2.1, 2.5] V  diode_IfVec=[.1, .2, .5, 1, 2, 4, 7, 10] A  diode_IrMat=[1e-06, 2e-06, 5e-06, 1e-05, 2.5e-05, 5e-05, .0001; 2e-06, 5e-06, 1e-05, 4e-05, 8e-05, .0002, .0005] A  diode_VrMat=[10, 100, 200, 250, 300, 325, 350; 10, 70, 160, 220, 270, 300, 320] V  diode_VrVec=[10, 20, 40, 50, 70, 80, 100] V  diode_IrVec=[1e-06, 2e-06, 5e-06, 1e-05, 2e-05, 5e-05, .0001] A  diode_Vr=-600 V  diode_Ls=150 nH  diode_Erec=0.03 J  diode_rec_loss_model=ee.enum.diode.reverseRecoveryModel.fixed  diode_ErecVal=0 J  diode_scaleWithIandV=true  diode_ErecMat=zeros(2, 3) J  diode_TjrecVec=[298.15, 398.15] K  diode_IfrecVec=[.1, 1, 10] A  diode_IrecVal=10 A  diode_VrecVal=10 V  diode_tFilter=1 / 1000 / 100 s  separateThermalPortForDiode=false  thermal_network_parameterization=ee.enum.thermalNetworkTopology.external  Rth=[.03, .2] K/W  Rth_Cauer=[.03, .1, .2] K/W  Rth_Foster=[.03, .2] K/W  thermal_mass_parameterization=ee.enum.thermalNetwork.timeconstant  thermal_mass=[3, 25] J/K  thermal_mass_Cauer=[3, 10, 25] J/K  thermal_mass_Foster=[33, 50] J/K  thermal_time_constant=[.1, 5] s  thermal_time_constant_Cauer=[.1, 1, 5] s  thermal_time_constant_Foster=[1, 10] s  thermal_mass_initial_temperatures=[25, 25] degC  thermal_mass_initial_temperatures_Cauer=[25, 25, 25] degC  junction_thermal_mass=0.1 J/K  Tvec_initial_Foster=[25, 25, 25, 25] degC  RthDiode=[.03, .2] K/W  RthCauerDiode=[.03, .1, .2] K/W  RthFosterDiode=[.03, .2] K/W  thermalMassDiode=[3, 25] J/K  thermalMassCauerDiode=[3, 10, 25] J/K  thermalMassFosterDiode=[33, 50] J/K  thermalTauDiode=[.1, 5] s  thermalTauCauerDiode=[.1, 1, 5] s  thermalTauFosterDiode=[1, 10] s  thermalMassInitTempDiode=[25, 25] degC  thermalMassInitTempCauerDiode=[25, 25, 25] degC  junctionthermalMassDiode=0.1 J/K  TVecInitialFosterDiode=[25, 25, 25, 25] degC  no_thermal_network=0  mosfet_junction_temperature_specify=off  mosfet_junction_temperature_priority=None  mosfet_junction_temperature=25 degC  mosfet_junction_temperature_nominal_specify=off  mosfet_junction_temperature_nominal_value=1  mosfet_junction_temperature_nominal_unit=degC  diode_junction_temperature_specify=off  diode_junction_temperature_priority=None  diode_junction_temperature=25 degC  diode_junction_temperature_nominal_specify=off  diode_junction_temperature_nominal_value=1  diode_junction_temperature_nominal_unit=degC  Qj_specify=off  Qj_priority=None  Qj=0 W  Qj_nominal_specify=off  Qj_nominal_value=1  Qj_nominal_unit=W  accumulatedSwitchingLosses_specify=off  accumulatedSwitchingLosses_priority=None  accumulatedSwitchingLosses=0 J
  CH (S5) : ee_lib/Semiconductors & Converters/MOSFET (Ideal, Switching)  port_option=ee.enum.controlport.ps  Rds=0.01 Ohm  Goff=1e-6 1/Ohm  Vth=0.5 V  diode_param=2  diode_Vf=0.1 V  diode_Ron=0.001 Ohm  diode_Goff=1e-5 1/Ohm  diode_C=50e-9 F  diode_iRM=-235 A  diode_iF=300 A  diode_idot=-50 A/us  diode_trr_param=1  diode_trr_factor=3  diode_trr=15 us  diode_Qrr=1500 s*uA  ids_specify=off  ids_priority=None  ids=0 A  ids_nominal_specify=off  ids_nominal_value=1  ids_nominal_unit=A  vds_specify=off  vds_priority=None  vds=0 V  vds_nominal_specify=off  vds_nominal_value=1  vds_nominal_unit=V  vgs_specify=off  vgs_priority=None  vgs=0 V  vgs_nominal_specify=off  vgs_nominal_value=1  vgs_nominal_unit=V  thermal_loss_option=2  Von_data=[0, 1.1, 1.3, 1.45, 1.75, 2.25, 2.7; 0, 1, 1.15, 1.35, 1.7, 2.35, 3] V  Tj=[298.15, 398.15] K  Iout_data=[0, 10, 50, 100, 200, 400, 600] A  Eon_data=[0, .29, 1.43, 2.86, 5.71, 13.14, 22.86; 0, .57, 2.63, 5.14, 10.29, 20.57, 30.29] * 1e-3 J  Eoff_data=[0, .21, 1.07, 2.14, 4.29, 9.86, 17.14; 0, .43, 1.97, 3.86, 7.71, 15.43, 22.71] * 1e-3 J  Eon_data_3D=[zeros(2, 5, 3)] J  Eoff_data_3D=[zeros(2, 5, 3)] J  Tj_loss=[298.15, 448.15] K  Iout_data_loss=[0, 10, 20, 30, 40] A  tabulateWithVds=false  Vds_loss=[0, 150, 300] V  Eon_scalar=22.86e-3 J  Eoff_scalar=17.14e-3 J  Voff=300 V  Iout_scalar=600 A  useCurrentFromPreviousCycle=false  useVoltageFromPreviousCycle=false  diodeModelType=ee.enum.converters.diodeModelType.pwl  diodeTableType=ee.enum.diode.tableType.IfMat  diode_ReverseIVType=ee.enum.diode.diodeReverseIV.constant  diode_IfMat=[.07, .12, .19, 1.75, 4.24, 7.32, 11.2; .16, .3, .72, 2.14, 4.02, 6.35, 9.12] A  diode_VfMat=[.9, 1.15, 1.25, 1.5, 1.75, 2.17, 2.6, 2.85; .58, .68, .75, 1.1, 1.38, 1.77, 2.27, 2.7] V  diode_TjVec=[25, 125] degC  diode_VfVec=[.5, .7, .9, 1.3, 1.7, 2.1, 2.5] V  diode_IfVec=[.1, .2, .5, 1, 2, 4, 7, 10] A  diode_IrMat=[1e-06, 2e-06, 5e-06, 1e-05, 2.5e-05, 5e-05, .0001; 2e-06, 5e-06, 1e-05, 4e-05, 8e-05, .0002, .0005] A  diode_VrMat=[10, 100, 200, 250, 300, 325, 350; 10, 70, 160, 220, 270, 300, 320] V  diode_VrVec=[10, 20, 40, 50, 70, 80, 100] V  diode_IrVec=[1e-06, 2e-06, 5e-06, 1e-05, 2e-05, 5e-05, .0001] A  diode_Vr=-600 V  diode_Ls=150 nH  diode_Erec=0.03 J  diode_rec_loss_model=ee.enum.diode.reverseRecoveryModel.fixed  diode_ErecVal=0 J  diode_scaleWithIandV=true  diode_ErecMat=zeros(2, 3) J  diode_TjrecVec=[298.15, 398.15] K  diode_IfrecVec=[.1, 1, 10] A  diode_IrecVal=10 A  diode_VrecVal=10 V  diode_tFilter=1 / 1000 / 100 s  separateThermalPortForDiode=false  thermal_network_parameterization=ee.enum.thermalNetworkTopology.external  Rth=[.03, .2] K/W  Rth_Cauer=[.03, .1, .2] K/W  Rth_Foster=[.03, .2] K/W  thermal_mass_parameterization=ee.enum.thermalNetwork.timeconstant  thermal_mass=[3, 25] J/K  thermal_mass_Cauer=[3, 10, 25] J/K  thermal_mass_Foster=[33, 50] J/K  thermal_time_constant=[.1, 5] s  thermal_time_constant_Cauer=[.1, 1, 5] s  thermal_time_constant_Foster=[1, 10] s  thermal_mass_initial_temperatures=[25, 25] degC  thermal_mass_initial_temperatures_Cauer=[25, 25, 25] degC  junction_thermal_mass=0.1 J/K  Tvec_initial_Foster=[25, 25, 25, 25] degC  RthDiode=[.03, .2] K/W  RthCauerDiode=[.03, .1, .2] K/W  RthFosterDiode=[.03, .2] K/W  thermalMassDiode=[3, 25] J/K  thermalMassCauerDiode=[3, 10, 25] J/K  thermalMassFosterDiode=[33, 50] J/K  thermalTauDiode=[.1, 5] s  thermalTauCauerDiode=[.1, 1, 5] s  thermalTauFosterDiode=[1, 10] s  thermalMassInitTempDiode=[25, 25] degC  thermalMassInitTempCauerDiode=[25, 25, 25] degC  junctionthermalMassDiode=0.1 J/K  TVecInitialFosterDiode=[25, 25, 25, 25] degC  no_thermal_network=0  mosfet_junction_temperature_specify=off  mosfet_junction_temperature_priority=None  mosfet_junction_temperature=25 degC  mosfet_junction_temperature_nominal_specify=off  mosfet_junction_temperature_nominal_value=1  mosfet_junction_temperature_nominal_unit=degC  diode_junction_temperature_specify=off  diode_junction_temperature_priority=None  diode_junction_temperature=25 degC  diode_junction_temperature_nominal_specify=off  diode_junction_temperature_nominal_value=1  diode_junction_temperature_nominal_unit=degC  Qj_specify=off  Qj_priority=None  Qj=0 W  Qj_nominal_specify=off  Qj_nominal_value=1  Qj_nominal_unit=W  accumulatedSwitchingLosses_specify=off  accumulatedSwitchingLosses_priority=None  accumulatedSwitchingLosses=0 J
  CL (S6) : ee_lib/Semiconductors & Converters/MOSFET (Ideal, Switching)  port_option=ee.enum.controlport.ps  Rds=0.01 Ohm  Goff=1e-6 1/Ohm  Vth=0.5 V  diode_param=2  diode_Vf=0.1 V  diode_Ron=0.001 Ohm  diode_Goff=1e-5 1/Ohm  diode_C=50e-9 F  diode_iRM=-235 A  diode_iF=300 A  diode_idot=-50 A/us  diode_trr_param=1  diode_trr_factor=3  diode_trr=15 us  diode_Qrr=1500 s*uA  ids_specify=off  ids_priority=None  ids=0 A  ids_nominal_specify=off  ids_nominal_value=1  ids_nominal_unit=A  vds_specify=off  vds_priority=None  vds=0 V  vds_nominal_specify=off  vds_nominal_value=1  vds_nominal_unit=V  vgs_specify=off  vgs_priority=None  vgs=0 V  vgs_nominal_specify=off  vgs_nominal_value=1  vgs_nominal_unit=V  thermal_loss_option=2  Von_data=[0, 1.1, 1.3, 1.45, 1.75, 2.25, 2.7; 0, 1, 1.15, 1.35, 1.7, 2.35, 3] V  Tj=[298.15, 398.15] K  Iout_data=[0, 10, 50, 100, 200, 400, 600] A  Eon_data=[0, .29, 1.43, 2.86, 5.71, 13.14, 22.86; 0, .57, 2.63, 5.14, 10.29, 20.57, 30.29] * 1e-3 J  Eoff_data=[0, .21, 1.07, 2.14, 4.29, 9.86, 17.14; 0, .43, 1.97, 3.86, 7.71, 15.43, 22.71] * 1e-3 J  Eon_data_3D=[zeros(2, 5, 3)] J  Eoff_data_3D=[zeros(2, 5, 3)] J  Tj_loss=[298.15, 448.15] K  Iout_data_loss=[0, 10, 20, 30, 40] A  tabulateWithVds=false  Vds_loss=[0, 150, 300] V  Eon_scalar=22.86e-3 J  Eoff_scalar=17.14e-3 J  Voff=300 V  Iout_scalar=600 A  useCurrentFromPreviousCycle=false  useVoltageFromPreviousCycle=false  diodeModelType=ee.enum.converters.diodeModelType.pwl  diodeTableType=ee.enum.diode.tableType.IfMat  diode_ReverseIVType=ee.enum.diode.diodeReverseIV.constant  diode_IfMat=[.07, .12, .19, 1.75, 4.24, 7.32, 11.2; .16, .3, .72, 2.14, 4.02, 6.35, 9.12] A  diode_VfMat=[.9, 1.15, 1.25, 1.5, 1.75, 2.17, 2.6, 2.85; .58, .68, .75, 1.1, 1.38, 1.77, 2.27, 2.7] V  diode_TjVec=[25, 125] degC  diode_VfVec=[.5, .7, .9, 1.3, 1.7, 2.1, 2.5] V  diode_IfVec=[.1, .2, .5, 1, 2, 4, 7, 10] A  diode_IrMat=[1e-06, 2e-06, 5e-06, 1e-05, 2.5e-05, 5e-05, .0001; 2e-06, 5e-06, 1e-05, 4e-05, 8e-05, .0002, .0005] A  diode_VrMat=[10, 100, 200, 250, 300, 325, 350; 10, 70, 160, 220, 270, 300, 320] V  diode_VrVec=[10, 20, 40, 50, 70, 80, 100] V  diode_IrVec=[1e-06, 2e-06, 5e-06, 1e-05, 2e-05, 5e-05, .0001] A  diode_Vr=-600 V  diode_Ls=150 nH  diode_Erec=0.03 J  diode_rec_loss_model=ee.enum.diode.reverseRecoveryModel.fixed  diode_ErecVal=0 J  diode_scaleWithIandV=true  diode_ErecMat=zeros(2, 3) J  diode_TjrecVec=[298.15, 398.15] K  diode_IfrecVec=[.1, 1, 10] A  diode_IrecVal=10 A  diode_VrecVal=10 V  diode_tFilter=1 / 1000 / 100 s  separateThermalPortForDiode=false  thermal_network_parameterization=ee.enum.thermalNetworkTopology.external  Rth=[.03, .2] K/W  Rth_Cauer=[.03, .1, .2] K/W  Rth_Foster=[.03, .2] K/W  thermal_mass_parameterization=ee.enum.thermalNetwork.timeconstant  thermal_mass=[3, 25] J/K  thermal_mass_Cauer=[3, 10, 25] J/K  thermal_mass_Foster=[33, 50] J/K  thermal_time_constant=[.1, 5] s  thermal_time_constant_Cauer=[.1, 1, 5] s  thermal_time_constant_Foster=[1, 10] s  thermal_mass_initial_temperatures=[25, 25] degC  thermal_mass_initial_temperatures_Cauer=[25, 25, 25] degC  junction_thermal_mass=0.1 J/K  Tvec_initial_Foster=[25, 25, 25, 25] degC  RthDiode=[.03, .2] K/W  RthCauerDiode=[.03, .1, .2] K/W  RthFosterDiode=[.03, .2] K/W  thermalMassDiode=[3, 25] J/K  thermalMassCauerDiode=[3, 10, 25] J/K  thermalMassFosterDiode=[33, 50] J/K  thermalTauDiode=[.1, 5] s  thermalTauCauerDiode=[.1, 1, 5] s  thermalTauFosterDiode=[1, 10] s  thermalMassInitTempDiode=[25, 25] degC  thermalMassInitTempCauerDiode=[25, 25, 25] degC  junctionthermalMassDiode=0.1 J/K  TVecInitialFosterDiode=[25, 25, 25, 25] degC  no_thermal_network=0  mosfet_junction_temperature_specify=off  mosfet_junction_temperature_priority=None  mosfet_junction_temperature=25 degC  mosfet_junction_temperature_nominal_specify=off  mosfet_junction_temperature_nominal_value=1  mosfet_junction_temperature_nominal_unit=degC  diode_junction_temperature_specify=off  diode_junction_temperature_priority=None  diode_junction_temperature=25 degC  diode_junction_temperature_nominal_specify=off  diode_junction_temperature_nominal_value=1  diode_junction_temperature_nominal_unit=degC  Qj_specify=off  Qj_priority=None  Qj=0 W  Qj_nominal_specify=off  Qj_nominal_value=1  Qj_nominal_unit=W  accumulatedSwitchingLosses_specify=off  accumulatedSwitchingLosses_priority=None  accumulatedSwitchingLosses=0 J
  Current Sensor (Three-Phase) : ee_lib/Sensors & Transducers/Current Sensor (Three-Phase)
      settings: InternalSimscapePortConfiguration="{\"Bottom\":[],\"Left\":[{\"id\":\"a1\",\"label\":\"a1\",\"type\":\"foundation.electrical.electrical\"},{\"id\":\"b1\",\"label\":\"b1\",\"type\":\"foundation.electrical.electrical\"},{\"id\":\"c1\",\"label\":\"c1\",\"type\":\"foundation.electrical.electrical\"}],\"Right\":[{\"id\":\"I_output\",\"label\":\"I\",\"type\":\"output\"},{\"id\":\"a2\",\"label\":\"a2\",\"type\":\"foundation.electrical.electrical\"},{\"id\":\"b2\",\"label\":\"b2\",\"type\":\"foundation.electrical.electrical\"},{\"id\":\"c2\",\"label\":\"c2\",\"type\":\"foundation.electrical.electrical\"}],\"Top\":[]}"
  Demux : Demux  Outputs=6
  Electrical Reference1 : fl_lib/Electrical/Electrical Elements/Electrical Reference
  PS-Simulink Converter : nesl_utility/PS-Simulink Converter  PhysicalDomain=network_engine_domain  SubClassName=ps_output  LeftPortType=input  RightPortType=output  PseudoPeriodic=off  Frequencies=[]  VectorFormat=1-D array  Unit=1  AffineConversion=off
  PS-Simulink Converter1 : nesl_utility/PS-Simulink Converter  PhysicalDomain=network_engine_domain  SubClassName=ps_output  LeftPortType=input  RightPortType=output  PseudoPeriodic=off  Frequencies=[]  VectorFormat=1-D array  Unit=1  AffineConversion=off
  Phase Voltage Sensor (Three-Phase) : ee_lib/Sensors & Transducers/Phase Voltage Sensor (Three-Phase)
      settings: InternalSimscapePortConfiguration="{\"Bottom\":[],\"Left\":[{\"id\":\"a1\",\"label\":\"a1\",\"type\":\"foundation.electrical.electrical\"},{\"id\":\"b1\",\"label\":\"b1\",\"type\":\"foundation.electrical.electrical\"},{\"id\":\"c1\",\"label\":\"c1\",\"type\":\"foundation.electrical.electrical\"}],\"Right\":[{\"id\":\"V_output\",\"label\":\"V\",\"type\":\"output\"},{\"id\":\"a2\",\"label\":\"a2\",\"type\":\"foundation.electrical.electrical\"},{\"id\":\"b2\",\"label\":\"b2\",\"type\":\"foundation.electrical.electrical\"},{\"id\":\"c2\",\"label\":\"c2\",\"type\":\"foundation.electrical.electrical\"}],\"Top\":[]}"
  Simulink-PS Converter{,1..5} (6 alike) : nesl_utility/Simulink-PS Converter  PhysicalDomain=network_engine_domain  SubClassName=ps_input  LeftPortType=input  RightPortType=output  PseudoPeriodic=off  Frequencies=[]  NoiseDistribution=none  NoiseParameters=[]  Unit=1  AffineConversion=off  FilteringAndDerivatives=provide  SimscapeFilterOrder=1  InputFilterTimeConstant=0.001  UdotUserProvided=0
  Three-phase currents : Scope
  Three-phase voltages : Scope
  Phase A : PMIOPort  Side=Right
  Phase B : PMIOPort  Port=2  Side=Right
  Phase C : PMIOPort  Port=3  Side=Right
  + : PMIOPort  Port=4  Side=Left
  - : PMIOPort  Port=5  Side=Left
  wires:
  [BH] -> Simulink-PS Converter2/1
  [CL] -> Simulink-PS Converter5/1
  Switching pattern/1 -> Demux/1
  Demux/1 -> [AH]
  [AH] -> Simulink-PS Converter/1
  [AL] -> Simulink-PS Converter1/1
  Demux/5 -> [CH]
  Demux/4 -> [BL]
  [BL] -> Simulink-PS Converter3/1
  Demux/3 -> [BH]
  [CH] -> Simulink-PS Converter4/1
  Demux/2 -> [AL]
  Demux/6 -> [CL]
  PS-Simulink Converter1/1 -> Three-phase voltages/1
  ? -> ?
  ? -> ?
  PS-Simulink Converter/1 -> Three-phase currents/1
  connections:
  CH (S5)/RConn1 -- BH (S3)/RConn1 -- AH (S1)/RConn1 -- +/RConn1
  Phase Voltage Sensor (Three-Phase)/RConn3 -- Phase Voltage Sensor (Three-Phase)/RConn4 -- Phase Voltage Sensor (Three-Phase)/RConn2 -- Electrical Reference1/LConn1
  Current Sensor (Three-Phase)/RConn3 -- Phase B/RConn1
  Simulink-PS Converter3/RConn1 -- BL (S4)/LConn1
  Current Sensor (Three-Phase)/RConn4 -- Phase C/RConn1
  AH (S1)/RConn2 -- Current Sensor (Three-Phase)/LConn1 -- Phase Voltage Sensor (Three-Phase)/LConn1 -- AL (S2)/RConn1
  AL (S2)/RConn2 -- CL (S6)/RConn2 -- BL (S4)/RConn2 -- -/RConn1
  BH (S3)/RConn2 -- Current Sensor (Three-Phase)/LConn2 -- Phase Voltage Sensor (Three-Phase)/LConn2 -- BL (S4)/RConn1
  Simulink-PS Converter5/RConn1 -- CL (S6)/LConn1
  CH (S5)/RConn2 -- Phase Voltage Sensor (Three-Phase)/LConn3 -- Current Sensor (Three-Phase)/LConn3 -- CL (S6)/RConn1
  Simulink-PS Converter4/RConn1 -- CH (S5)/LConn1
  PS-Simulink Converter1/LConn1 -- Phase Voltage Sensor (Three-Phase)/RConn1
  Simulink-PS Converter/RConn1 -- AH (S1)/LConn1
  Current Sensor (Three-Phase)/RConn2 -- Phase A/RConn1
  Simulink-PS Converter1/RConn1 -- AL (S2)/LConn1
  Simulink-PS Converter2/RConn1 -- BH (S3)/LConn1
  PS-Simulink Converter/LConn1 -- Current Sensor (Three-Phase)/RConn1
